simulink library "casper_library_scopes"  (Simulink 8.0)
settings: Solver=ode45  SolverMode=SingleTasking  StartTime=0.0  StopTime=10.0  RelTol=1e-3
libraries: xbsIndex_r4 x476, xps_library x33, casper_library_misc x13, casper_library_scopes x5, casper_library_flow_control x1, simulink x1
(part 2 of 5)

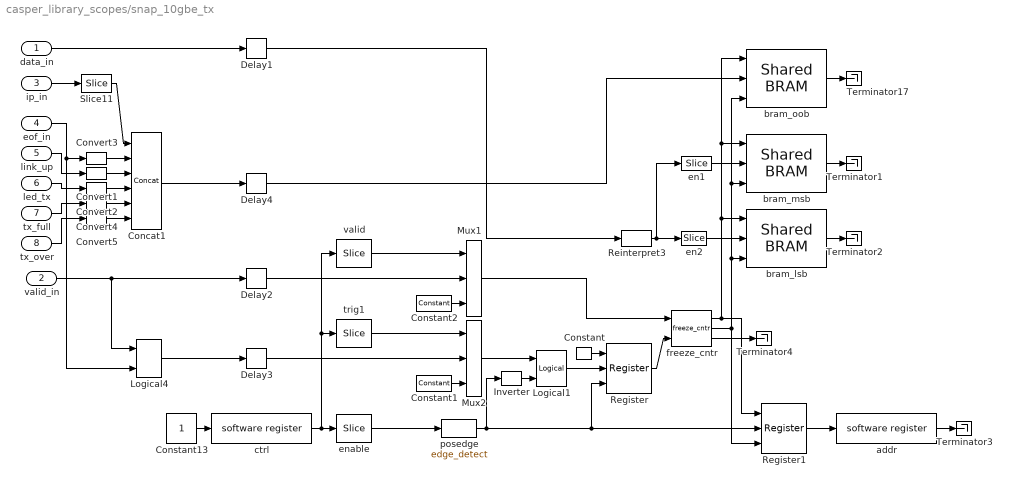
== system casper_library_scopes/snap_10gbe_tx ==
  data_in : Inport
  valid_in : Inport  Port=2
  ip_in : Inport  Port=3
  eof_in : Inport  Port=4
  link_up : Inport  Port=5
  led_tx : Inport  Port=6
  tx_full : Inport  Port=7
  tx_over : Inport  Port=8
  Concat1 : xbsIndex_r4/Concat  num_inputs=6  dbl_ovrd=off  block_type=concat
      settings: block_version=10.1.3
  Constant : xbsIndex_r4/Constant  const=1  gui_display_data_type=Fixed-point  arith_type=Boolean  n_bits=1  bin_pt=0  preci_type=Single  exp_width=8  frac_width=24  explicit_period=on  period=1  equ=P=C  opselect=C  inp2=PCIN>>17  opr=+  inp1=P  carry=CIN  dbl_ovrd=off  block_type=constant
  Constant1 : xbsIndex_r4/Constant  const=1  gui_display_data_type=Fixed-point  arith_type=Boolean  n_bits=1  bin_pt=0  preci_type=Single  exp_width=8  frac_width=24  explicit_period=on  period=1  equ=P=C  opselect=C  inp2=PCIN>>17  opr=+  inp1=P  carry=CIN  dbl_ovrd=off  block_type=constant
  Constant13 : Constant
  Constant2 : xbsIndex_r4/Constant  const=1  gui_display_data_type=Fixed-point  arith_type=Boolean  n_bits=1  bin_pt=0  preci_type=Single  exp_width=8  frac_width=24  explicit_period=on  period=1  equ=P=C  opselect=C  inp2=PCIN>>17  opr=+  inp1=P  carry=CIN  dbl_ovrd=off  block_type=constant
  Convert{1..5} (5 alike) : xbsIndex_r4/Convert  gui_display_data_type=Fixed-point  arith_type=Unsigned  n_bits=1  bin_pt=0  float_type=Single  exp_bits=8  fraction_bits=24  quantization=Truncate  overflow=Wrap  en=off  latency=0  dbl_ovrd=off  pipeline=off  block_type=convert
      settings: xl_area=[0, 0, 0, 0, 0, 0, 0]  block_version=10.1.3
  Delay{1..4} (4 alike) : xbsIndex_r4/Delay  rst=off  infoeditControl=Selection of Reset will increase slice count due to use of real FFs and instead of SRLs  en=off  latency=2  dbl_ovrd=off  reg_retiming=on  block_type=delay
      settings: xl_area=[0, 0, 0, 0, 0, 0, 0]
  Inverter : xbsIndex_r4/Inverter  en=off  latency=0  dbl_ovrd=off  block_type=inv
      settings: xl_area=[0, 0, 0, 0, 0, 0, 0]
  Logical1 : xbsIndex_r4/Logical  logical_function=AND  inputs=2  en=off  latency=0  precision=Full  arith_type=Unsigned  n_bits=8  bin_pt=2  align_bp=on  dbl_ovrd=off  block_type=logical
      settings: xl_area=[0, 0, 0, 0, 0, 0, 0]
  Logical4 : xbsIndex_r4/Logical  logical_function=AND  inputs=2  en=off  latency=0  precision=Full  arith_type=Unsigned  n_bits=8  bin_pt=2  align_bp=on  dbl_ovrd=off  block_type=logical
      settings: xl_area=[0, 0, 0, 0, 0, 0, 0]
  Mux1 : xbsIndex_r4/Mux  inputs=2  en=off  latency=0  precision=Full  arith_type="Signed  (2's comp)"  n_bits=8  bin_pt=2  quantization=Truncate  overflow=Wrap  dbl_ovrd=off  block_type=mux
      settings: xl_area=[0, 0, 0, 0, 0, 0, 0]
  Mux2 : xbsIndex_r4/Mux  inputs=2  en=off  latency=0  precision=Full  arith_type="Signed  (2's comp)"  n_bits=8  bin_pt=2  quantization=Truncate  overflow=Wrap  dbl_ovrd=off  block_type=mux
      settings: xl_area=[0, 0, 0, 0, 0, 0, 0]
  Register : xbsIndex_r4/Register  init=0  rst=on  en=on  dbl_ovrd=off  block_type=register
      settings: xl_area=[0, 0, 0, 0, 0, 0, 0]
  Register1 : xbsIndex_r4/Register  init=0  rst=on  en=on  dbl_ovrd=off  block_type=register
      settings: xl_area=[0, 0, 0, 0, 0, 0, 0]
  Reinterpret3 : xbsIndex_r4/Reinterpret  force_arith_type=on  arith_type=Unsigned  force_bin_pt=on  bin_pt=0  block_type=reinterpret
      settings: infoedit="Changes signal type without altering the binary representation.   You can changed the signal between signed and unsigned, and relocate the binary point.<P><P>Hardware notes: In hardware this block costs nothing.<P><P>Example:  Suppose the input is 6 bits wide, signed, with 2 fractional bits, and the output is forced to unsigned with 0 fractional bits.  Then an input of -2.0 (1110.00 in binary 2's complement) becomes an output of 56 (111000 in binary)."  block_version=10.1.3
  Slice11 : xbsIndex_r4/Slice  nbits=32-5  boolean_output=off  mode=Lower Bit Location + Width  bit1=0  base1=MSB of Input  bit0=0  base0=LSB of Input  dbl_ovrd=off  block_type=slice
      settings: infoedit="Extracts a given range of bits from each input sample and presents it at the output.  The output type is ordinarily unsigned with binary point at zero, but can be Boolean when the slice is one bit wide.<P><P>Hardware notes: In hardware this block costs nothing."  block_version=10.1.3
  Terminator{1..4,17} (5 alike) : Terminator
  addr : xps_library/software register  Tag=xps:sw_reg  numios=1  io_dir=To Processor  io_delay=0  sample_period=1  name1=reg  bitwidth1=32  arith_type1=Unsigned  bin_pt1=0
  bram_lsb : xps_library/Shared BRAM  Tag=xps:bram  arith_type=Unsigned  addr_width=nsamples  data_width=32  reg_prim_output=on  reg_core_output=on  optimization=Minimum_Area  data_bin_pt=0  init_vals=0  sample_rate=1
  bram_msb : xps_library/Shared BRAM  Tag=xps:bram  arith_type=Unsigned  addr_width=nsamples  data_width=32  reg_prim_output=on  reg_core_output=on  optimization=Minimum_Area  data_bin_pt=0  init_vals=0  sample_rate=1
  bram_oob : xps_library/Shared BRAM  Tag=xps:bram  arith_type=Unsigned  addr_width=nsamples  data_width=32  reg_prim_output=on  reg_core_output=on  optimization=Minimum_Area  data_bin_pt=0  init_vals=0  sample_rate=1
  ctrl : xps_library/software register  Tag=xps:sw_reg  numios=1  io_dir=From Processor  io_delay=0  sample_period=1  name1=reg  bitwidth1=32  arith_type1=Unsigned  bin_pt1=0
  en1 : xbsIndex_r4/Slice  nbits=32  boolean_output=off  mode=Lower Bit Location + Width  bit1=0  base1=LSB of Input  bit0=32  base0=LSB of Input  dbl_ovrd=off  block_type=slice
      settings: infoedit="Extracts a given range of bits from each input sample and presents it at the output.  The output type is ordinarily unsigned with binary point at zero, but can be Boolean when the slice is one bit wide.<P><P>Hardware notes: In hardware this block costs nothing."  block_version=10.1.3
  en2 : xbsIndex_r4/Slice  nbits=32  boolean_output=off  mode=Lower Bit Location + Width  bit1=0  base1=LSB of Input  bit0=0  base0=LSB of Input  dbl_ovrd=off  block_type=slice
      settings: infoedit="Extracts a given range of bits from each input sample and presents it at the output.  The output type is ordinarily unsigned with binary point at zero, but can be Boolean when the slice is one bit wide.<P><P>Hardware notes: In hardware this block costs nothing."  block_version=10.1.3
  enable : xbsIndex_r4/Slice  nbits=1  boolean_output=on  mode=Lower Bit Location + Width  bit1=0  base1=LSB of Input  bit0=0  base0=LSB of Input  dbl_ovrd=off  block_type=slice
      settings: infoedit="Extracts a given range of bits from each input sample and presents it at the output.  The output type is ordinarily unsigned with binary point at zero, but can be Boolean when the slice is one bit wide.<P><P>Hardware notes: In hardware this block costs nothing."  block_version=10.1.3
  freeze_cntr : casper_library_misc/freeze_cntr  CounterBits=nsamples
  posedge : casper_library_misc/edge_detect  edge=Rising  polarity=Active High  x_in=[0 0.08 0.08 0.16 0.16 0.24 0.24 0.32 0.32 0.4]  y_in="[-1 -1  1  1  1  1  1  1  1  1]"  x_out=[0.6 0.68 0.68 0.76 0.76 0.84 0.84 0.92 0.92 1]  y_out="[-1 -1  1  1 -1 -1 -1 -1 -1 -1]"
  trig1 : xbsIndex_r4/Slice  nbits=1  boolean_output=on  mode=Lower Bit Location + Width  bit1=0  base1=LSB of Input  bit0=1  base0=LSB of Input  dbl_ovrd=off  block_type=slice
      settings: infoedit="Extracts a given range of bits from each input sample and presents it at the output.  The output type is ordinarily unsigned with binary point at zero, but can be Boolean when the slice is one bit wide.<P><P>Hardware notes: In hardware this block costs nothing."  block_version=10.1.3
  valid : xbsIndex_r4/Slice  nbits=1  boolean_output=on  mode=Lower Bit Location + Width  bit1=0  base1=LSB of Input  bit0=2  base0=LSB of Input  dbl_ovrd=off  block_type=slice
      settings: infoedit="Extracts a given range of bits from each input sample and presents it at the output.  The output type is ordinarily unsigned with binary point at zero, but can be Boolean when the slice is one bit wide.<P><P>Hardware notes: In hardware this block costs nothing."  block_version=10.1.3
  wires:
  freeze_cntr/3 -> Terminator4/1
  addr/1 -> Terminator3/1
  bram_lsb/1 -> Terminator2/1
  bram_msb/1 -> Terminator1/1
  bram_oob/1 -> Terminator17/1
  Convert5/1 -> Concat1/6
  Convert4/1 -> Concat1/5
  Convert2/1 -> Concat1/4
  Convert1/1 -> Concat1/3
  Convert3/1 -> Concat1/2
  tx_over/1 -> Convert5/1
  tx_full/1 -> Convert4/1
  led_tx/1 -> Convert2/1
  link_up/1 -> Convert1/1
  eof_in/1 -> Logical4/2, Convert3/1
  Delay3/1 -> Mux2/2
  Delay2/1 -> Mux1/2
  valid_in/1 -> Logical4/1, Delay2/1
  Logical4/1 -> Delay3/1
  Delay4/1 -> bram_oob/2
  Delay1/1 -> Reinterpret3/1
  ip_in/1 -> Slice11/1
  data_in/1 -> Delay1/1
  Concat1/1 -> Delay4/1
  Slice11/1 -> Concat1/1
  freeze_cntr/1 -> bram_lsb/1, bram_msb/1, bram_oob/1, Register1/1
  Register/1 -> freeze_cntr/2
  Mux2/1 -> Logical1/1
  Inverter/1 -> Logical1/2
  Logical1/1 -> Register/2
  valid/1 -> Mux1/1
  trig1/1 -> Mux2/1
  Register1/1 -> addr/1
  Constant2/1 -> Mux1/3
  Mux1/1 -> freeze_cntr/1
  Constant1/1 -> Mux2/3
  Constant/1 -> Register/1
  posedge/1 -> Inverter/1, Register1/2, Register/3
  ctrl/1 -> trig1/1, valid/1, enable/1
  Constant13/1 -> ctrl/1
  freeze_cntr/2 -> bram_lsb/3, bram_msb/3, bram_oob/3, Register1/3
  enable/1 -> posedge/1
  Reinterpret3/1 -> en1/1, en2/1
  en1/1 -> bram_msb/2
  en2/1 -> bram_lsb/2

== system casper_library_scopes/snap_32n ==
  trig : Inport
  din : Inport  Port=2
  Constant : Constant  Value=0
  read_freeze : xps_library/software register  Tag=xps:sw_reg  numios=1  io_dir=From Processor  io_delay=0  sample_period=1  name1=reg  bitwidth1=32  arith_type1=Unsigned  bin_pt1=0
  sc0 : casper_library_scopes/sc  nsamples=11  offset=0
  sc1 : casper_library_scopes/sc  nsamples=11  offset=32
  sc2 : casper_library_scopes/sc  nsamples=11  offset=64
  sc3 : casper_library_scopes/sc  nsamples=11  offset=96
  wires:
  Constant/1 -> read_freeze/1
  trig/1 -> sc0/2, sc1/2, sc2/2, sc3/2
  din/1 -> sc0/1, sc1/1, sc2/1, sc3/1
  read_freeze/1 -> sc0/3, sc1/3, sc2/3, sc3/3

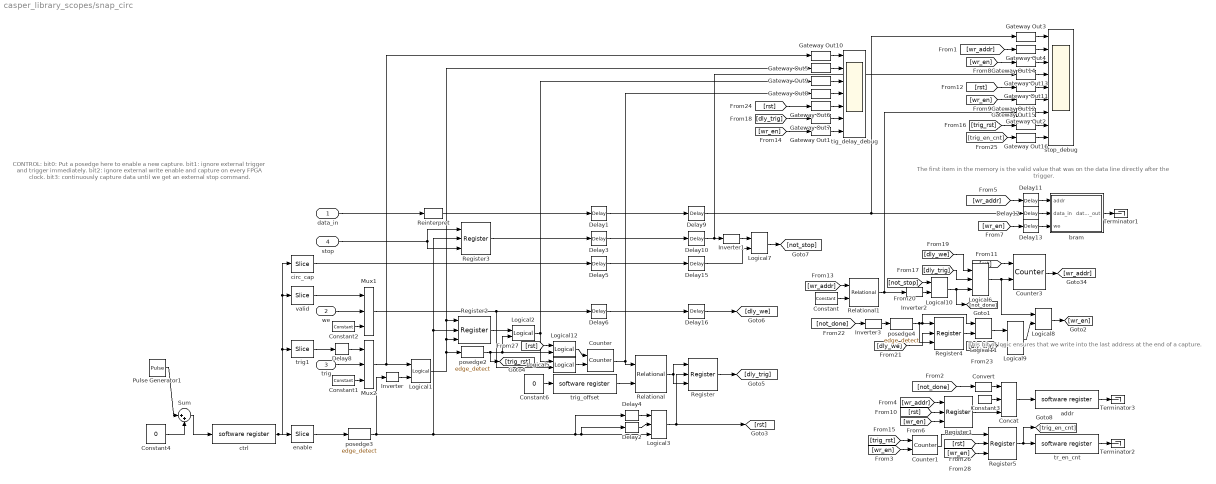
== system casper_library_scopes/snap_circ ==
  note: This bit of logic ensures that we
      | write into the last address
      | at the end of a capture.
  note: The first item in the memory
      | is the valid value that was on the
      | data line directly after the trigger.
  note: CONTROL:
      | bit0: Put a posedge here to enable a new capture.
      | bit1: ignore external trigger and trigger immediately.
      | bit2: ignore external write enable and capture on every FPGA clock.
      | bit3: continuously capture data until we get an external stop command.
  data_in : Inport
  we : Inport  Port=2
  trig : Inport  Port=3
  stop : Inport  Port=4
  Concat : xbsIndex_r4/Concat  num_inputs=3  dbl_ovrd=off  block_type=concat
      settings: block_version=10.1.3
  Constant : xbsIndex_r4/Constant  const=(2^nsamples)-1  gui_display_data_type=Fixed-point  arith_type=Unsigned  n_bits=nsamples  bin_pt=0  preci_type=Single  exp_width=8  frac_width=24  explicit_period=on  period=1  equ=P=C  opselect=C  inp2=PCIN>>17  opr=+  inp1=P  carry=CIN  dbl_ovrd=off  block_type=constant
  Constant1 : xbsIndex_r4/Constant  const=1  gui_display_data_type=Fixed-point  arith_type=Boolean  n_bits=1  bin_pt=0  preci_type=Single  exp_width=8  frac_width=24  explicit_period=on  period=1  equ=P=C  opselect=C  inp2=PCIN>>17  opr=+  inp1=P  carry=CIN  dbl_ovrd=off  block_type=constant
  Constant2 : xbsIndex_r4/Constant  const=1  gui_display_data_type=Fixed-point  arith_type=Boolean  n_bits=1  bin_pt=0  preci_type=Single  exp_width=8  frac_width=24  explicit_period=on  period=1  equ=P=C  opselect=C  inp2=PCIN>>17  opr=+  inp1=P  carry=CIN  dbl_ovrd=off  block_type=constant
  Constant3 : xbsIndex_r4/Constant  const=0  gui_display_data_type=Fixed-point  arith_type=Unsigned  n_bits=32-nsamples-1  bin_pt=0  preci_type=Single  exp_width=8  frac_width=24  explicit_period=on  period=1  equ=P=C  opselect=C  inp2=PCIN>>17  opr=+  inp1=P  carry=CIN  dbl_ovrd=off  block_type=constant
  Constant4 : Constant  Value=0
  Constant6 : Constant  Value=0
  Convert : xbsIndex_r4/Convert  gui_display_data_type=Fixed-point  arith_type=Unsigned  n_bits=1  bin_pt=0  float_type=Single  exp_bits=8  fraction_bits=24  quantization=Truncate  overflow=Wrap  en=off  latency=0  dbl_ovrd=off  pipeline=off  block_type=convert
      settings: block_version=10.1.3
  Counter : xbsIndex_r4/Counter  cnt_type=Free Running  cnt_to=Inf  operation=Up  start_count=0  cnt_by_val=1  arith_type=Unsigned  n_bits=32  bin_pt=0  load_pin=off  rst=on  en=on  explicit_period=on  period=1  dbl_ovrd=off  use_behavioral_HDL=off  implementation=Fabric  use_rpm=on  block_type=counter
      settings: xl_area=[0, 0, 0, 0, 0, 0, 0]
  Counter1 : xbsIndex_r4/Counter  cnt_type=Free Running  cnt_to=Inf  operation=Up  start_count=0  cnt_by_val=1  arith_type=Unsigned  n_bits=32  bin_pt=0  load_pin=off  rst=on  en=on  explicit_period=on  period=1  dbl_ovrd=off  use_behavioral_HDL=off  implementation=Fabric  use_rpm=on  block_type=counter
      settings: xl_area=[0, 0, 0, 0, 0, 0, 0]
  Counter3 : xbsIndex_r4/Counter  cnt_type=Free Running  cnt_to=1  operation=Up  start_count=0  cnt_by_val=1  arith_type=Unsigned  n_bits=nsamples  bin_pt=0  load_pin=off  rst=on  en=on  explicit_period=on  period=1  dbl_ovrd=off  use_behavioral_HDL=off  implementation=Fabric  use_rpm=on  block_type=counter
      settings: xl_area=[0, 0, 0, 0, 0, 0, 0]
  Delay{1,3..6,9..13,15..16} (12 alike) : xbsIndex_r4/Delay  rst=off  infoeditControl=Selection of Reset will increase slice count due to use of real FFs and instead of SRLs  en=off  latency=1  dbl_ovrd=off  reg_retiming=on  block_type=delay
      settings: xl_area=[0, 0, 0, 0, 0, 0, 0]
  Delay2 : xbsIndex_r4/Delay  rst=off  infoeditControl=Selection of Reset will increase slice count due to use of real FFs and instead of SRLs  en=off  latency=2  dbl_ovrd=off  reg_retiming=on  block_type=delay
      settings: xl_area=[0, 0, 0, 0, 0, 0, 0]
  Delay8 : xbsIndex_r4/Delay  rst=off  infoeditControl=Selection of Reset will increase slice count due to use of real FFs and instead of SRLs  en=off  latency=3  dbl_ovrd=off  reg_retiming=on  block_type=delay
      settings: xl_area=[0, 0, 0, 0, 0, 0, 0]
  Gateway Out{1..16} (16 alike) : xbsIndex_r4/Gateway Out  inherit_from_input=off  hdl_port=off  timing_constraint=None  locs_specified=off  LOCs={}  UseAsDAC=off  DACChannel='1'  block_type=gatewayout
      settings: infoedit="Gateway out block.  Converts Xilinx fixed point inputs into ouputs of type Simulink integer, double, or fixed point.<P><P>Hardware notes:  In hardware these blocks become top level output ports or are discarded, depending on how they are configured."  xl_area=[0, 0, 0, 0, 0, 0, 0]  block_version=10.1.3
  Inverter{,1..3} (4 alike) : xbsIndex_r4/Inverter  en=off  latency=0  dbl_ovrd=off  block_type=inv
      settings: xl_area=[0, 0, 0, 0, 0, 0, 0]
  Logical{1,5,7,9} (4 alike) : xbsIndex_r4/Logical  logical_function=AND  inputs=2  en=off  latency=0  precision=Full  arith_type=Unsigned  n_bits=8  bin_pt=2  align_bp=on  dbl_ovrd=off  block_type=logical
      settings: xl_area=[0, 0, 0, 0, 0, 0, 0]
  Logical{2,8,10..12} (5 alike) : xbsIndex_r4/Logical  logical_function=OR  inputs=2  en=off  latency=0  precision=Full  arith_type=Unsigned  n_bits=8  bin_pt=2  align_bp=on  dbl_ovrd=off  block_type=logical
      settings: xl_area=[0, 0, 0, 0, 0, 0, 0]
  Logical3 : xbsIndex_r4/Logical  logical_function=OR  inputs=3  en=off  latency=0  precision=Full  arith_type=Unsigned  n_bits=8  bin_pt=2  align_bp=on  dbl_ovrd=off  block_type=logical
      settings: xl_area=[0, 0, 0, 0, 0, 0, 0]
  Logical6 : xbsIndex_r4/Logical  logical_function=AND  inputs=3  en=off  latency=0  precision=Full  arith_type=Unsigned  n_bits=8  bin_pt=2  align_bp=on  dbl_ovrd=off  block_type=logical
      settings: xl_area=[0, 0, 0, 0, 0, 0, 0]
  Mux1 : xbsIndex_r4/Mux  inputs=2  en=off  latency=0  precision=Full  arith_type="Signed  (2's comp)"  n_bits=8  bin_pt=2  quantization=Truncate  overflow=Wrap  dbl_ovrd=off  block_type=mux
      settings: xl_area=[0, 0, 0, 0, 0, 0, 0]
  Mux2 : xbsIndex_r4/Mux  inputs=2  en=off  latency=0  precision=Full  arith_type="Signed  (2's comp)"  n_bits=8  bin_pt=2  quantization=Truncate  overflow=Wrap  dbl_ovrd=off  block_type=mux
      settings: xl_area=[0, 0, 0, 0, 0, 0, 0]
  Pulse Generator1 : DiscretePulseGenerator  Period=2^(nsamples+2)  PulseWidth=2
  Register{,1..5} (6 alike) : xbsIndex_r4/Register  init=0  rst=on  en=on  dbl_ovrd=off  block_type=register
      settings: xl_area=[0, 0, 0, 0, 0, 0, 0]
  Reinterpret : xbsIndex_r4/Reinterpret  force_arith_type=on  arith_type=Unsigned  force_bin_pt=on  bin_pt=0  block_type=reinterpret
      settings: infoedit="Changes signal type without altering the binary representation.   You can changed the signal between signed and unsigned, and relocate the binary point.<P><P>Hardware notes: In hardware this block costs nothing.<P><P>Example:  Suppose the input is 6 bits wide, signed, with 2 fractional bits, and the output is forced to unsigned with 0 fractional bits.  Then an input of -2.0 (1110.00 in binary 2's complement) becomes an output of 56 (111000 in binary)."  block_version=10.1.3
  Relational : xbsIndex_r4/Relational  mode=a>b  en=off  latency=0  dbl_ovrd=off  block_type=relational
      settings: xl_area=[0, 0, 0, 0, 0, 0, 0]  block_version=10.1.3
  Relational1 : xbsIndex_r4/Relational  mode=a>=b  en=off  latency=0  dbl_ovrd=off  block_type=relational
      settings: xl_area=[0, 0, 0, 0, 0, 0, 0]  block_version=10.1.3
  Sum : Sum  Inputs=|++
  Terminator1 : Terminator
  Terminator2 : Terminator
  Terminator3 : Terminator
  addr : xps_library/software register  Tag=xps:sw_reg  mode=one value  io_dir=To Processor  io_delay=0  sample_period=1  names=reg  bitwidths=32  arith_types=0  bin_pts=0  show_format=off
      settings: AttributesFormatString=1output
  bram : Subsystem  Tag=xps:bram  AncestorBlock=xps_library/Shared BRAM  mask{arith_type=Unsigned, addr_width=nsamples, data_width=32, reg_prim_output=on, reg_core_output=on, optimization=Minimum_Area, data_bin_pt=0, init_vals=0, sample_rate=1}
      mask prompts: arith_type "Output Data Type"; addr_width "Address width"; data_width "Data Width"; reg_prim_output "Register Primitive Output"; reg_core_output "Register Core Output"; data_bin_pt "Data Binary Point"; init_vals "Initial values (simulation only)"; sample_rate "Sample rate"
      mask init:
      | shared_bram_mask;
      mask TypeOptions arith_type: Unsigned | Signed  (2's comp)
      mask TypeOptions data_width: 8 | 16 | 32 | 64 | 128
      mask TypeOptions optimization: Minimum_Area | Low_Power
  circ_cap : xbsIndex_r4/Slice  nbits=1  boolean_output=on  mode=Lower Bit Location + Width  bit1=0  base1=LSB of Input  bit0=3  base0=LSB of Input  dbl_ovrd=off  block_type=slice
      settings: infoedit="Extracts a given range of bits from each input sample and presents it at the output.  The output type is ordinarily unsigned with binary point at zero, but can be Boolean when the slice is one bit wide.<P><P>Hardware notes: In hardware this block costs nothing."  block_version=10.1.3
  ctrl : xps_library/software register  Tag=xps:sw_reg  mode=one value  io_dir=From Processor  io_delay=0  sample_period=1  names=reg  bitwidths=32  arith_types=0  bin_pts=0  show_format=off
      settings: AttributesFormatString=1input
  enable : xbsIndex_r4/Slice  nbits=1  boolean_output=on  mode=Lower Bit Location + Width  bit1=0  base1=LSB of Input  bit0=0  base0=LSB of Input  dbl_ovrd=off  block_type=slice
      settings: infoedit="Extracts a given range of bits from each input sample and presents it at the output.  The output type is ordinarily unsigned with binary point at zero, but can be Boolean when the slice is one bit wide.<P><P>Hardware notes: In hardware this block costs nothing."  block_version=10.1.3
  posedge2 : casper_library_misc/edge_detect  edge=Rising  polarity=Active High  x_in=[0 0.08 0.08 0.16 0.16 0.24 0.24 0.32 0.32 0.4]  y_in="[-1 -1  1  1  1  1  1  1  1  1]"  x_out=[0.6 0.68 0.68 0.76 0.76 0.84 0.84 0.92 0.92 1]  y_out="[-1 -1  1  1 -1 -1 -1 -1 -1 -1]"
  posedge3 : casper_library_misc/edge_detect  edge=Rising  polarity=Active High  x_in=[0 0.08 0.08 0.16 0.16 0.24 0.24 0.32 0.32 0.4]  y_in="[-1 -1  1  1  1  1  1  1  1  1]"  x_out=[0.6 0.68 0.68 0.76 0.76 0.84 0.84 0.92 0.92 1]  y_out="[-1 -1  1  1 -1 -1 -1 -1 -1 -1]"
  posedge4 : casper_library_misc/edge_detect  edge=Rising  polarity=Active High  x_in=[0 0.08 0.08 0.16 0.16 0.24 0.24 0.32 0.32 0.4]  y_in="[-1 -1  1  1  1  1  1  1  1  1]"  x_out=[0.6 0.68 0.68 0.76 0.76 0.84 0.84 0.92 0.92 1]  y_out="[-1 -1  1  1 -1 -1 -1 -1 -1 -1]"
  stop_debug : Scope  NumInputPorts=9
      settings: YMin=2.72014e+008~0~0~-5~-5~-5~-5~-5~-5  YMax=3.00648e+008~110~1~5~5~5~5~5~5  SaveName=ScopeData12
  tig_delay_debug : Scope  NumInputPorts=7
      settings: YMin=2.72014e+008~0~0~-5~-5~-5~-5  YMax=3.00648e+008~110~1~5~5~5~5  SaveName=ScopeData16
  tr_en_cnt : xps_library/software register  Tag=xps:sw_reg  mode=one value  io_dir=To Processor  io_delay=0  sample_period=1  names=reg  bitwidths=32  arith_types=0  bin_pts=0  show_format=off
      settings: AttributesFormatString=1output
  trig1 : xbsIndex_r4/Slice  nbits=1  boolean_output=on  mode=Lower Bit Location + Width  bit1=0  base1=LSB of Input  bit0=1  base0=LSB of Input  dbl_ovrd=off  block_type=slice
      settings: infoedit="Extracts a given range of bits from each input sample and presents it at the output.  The output type is ordinarily unsigned with binary point at zero, but can be Boolean when the slice is one bit wide.<P><P>Hardware notes: In hardware this block costs nothing."  block_version=10.1.3
  trig_offset : xps_library/software register  Tag=xps:sw_reg  mode=one value  io_dir=From Processor  io_delay=0  sample_period=1  names=reg  bitwidths=32  arith_types=0  bin_pts=0  show_format=off
      settings: AttributesFormatString=1input
  valid : xbsIndex_r4/Slice  nbits=1  boolean_output=on  mode=Lower Bit Location + Width  bit1=0  base1=LSB of Input  bit0=2  base0=LSB of Input  dbl_ovrd=off  block_type=slice
      settings: infoedit="Extracts a given range of bits from each input sample and presents it at the output.  The output type is ordinarily unsigned with binary point at zero, but can be Boolean when the slice is one bit wide.<P><P>Hardware notes: In hardware this block costs nothing."  block_version=10.1.3
  wires:
  Delay6/1 -> Delay16/1
  Delay5/1 -> Delay15/1
  Delay3/1 -> Delay10/1
  Delay1/1 -> Delay9/1
  posedge2/1 -> [trig_rst], Logical12/2, Logical2/2
  [rst] -> Logical12/1
  Logical12/1 -> Counter/1
  Register5/1 -> [trig_en_cnt], tr_en_cnt/1
  [rst] -> Register5/2
  [wr_en] -> Register5/3
  Counter1/1 -> Register5/1
  Gateway Out16/1 -> stop_debug/9
  [trig_en_cnt] -> Gateway Out16/1
  Delay8/1 -> Mux2/1
  [rst] -> Gateway Out6/1
  Register4/1 -> Logical11/2
  Logical11/1 -> Logical9/1
  Logical9/1 -> Logical8/2
  [dly_we] -> Logical9/2
  [dly_we] -> Register4/2
  posedge4/1 -> Logical11/1, Register4/1, Register4/3
  Inverter3/1 -> posedge4/1
  [not_done] -> Inverter3/1
  Logical8/1 -> [wr_en]
  [not_stop] -> Logical10/1
  Logical7/1 -> [not_stop]
  [dly_trig] -> Logical6/2
  [dly_we] -> Logical6/1
  Delay16/1 -> [dly_we]
  [dly_trig] -> Gateway Out7/1
  Register/1 -> [dly_trig]
  [trig_rst] -> Gateway Out15/1
  Gateway Out15/1 -> stop_debug/8
  [trig_rst] -> Counter1/1
  [wr_en] -> Gateway Out1/1
  [wr_addr] -> Relational1/1
  Relational1/1 -> Inverter2/1, Gateway Out2/1
  [rst] -> Gateway Out11/1
  [rst] -> Counter3/1
  [rst] -> Register1/2
  [wr_en] -> Gateway Out12/1
  [wr_en] -> Gateway Out14/1
  [wr_en] -> Delay13/1
  [wr_en] -> Register1/3
  [wr_addr] -> Register1/1
  [wr_en] -> Counter1/2
  [not_done] -> Convert/1
  [wr_addr] -> Gateway Out4/1
  [wr_addr] -> Delay11/1
  Register1/1 -> Concat/3
  Logical5/1 -> Counter/2
  Delay15/1 -> Logical7/2
  Delay10/1 -> Gateway Out13/1, Inverter1/1
  Delay9/1 -> Gateway Out3/1, Delay12/1
  bram/1(data_out) -> Terminator1/1
  addr/1 -> Terminator3/1
  tr_en_cnt/1 -> Terminator2/1
  Constant3/1 -> Concat/2
  Convert/1 -> Concat/1
  circ_cap/1 -> Delay5/1
  stop/1 -> Register3/3, Register3/1
  Concat/1 -> addr/1
  Delay13/1 -> bram/3(we)
  Delay12/1 -> bram/2(data_in)
  Delay11/1 -> bram/1(addr)
  Inverter2/1 -> Logical10/2
  Logical10/1 -> [not_done], Logical6/3
  Logical3/1 -> [rst], Register/2
  Gateway Out2/1 -> stop_debug/7
  Gateway Out12/1 -> stop_debug/6
  Gateway Out3/1 -> stop_debug/1
  Gateway Out11/1 -> stop_debug/5
  Gateway Out13/1 -> stop_debug/4
  Gateway Out4/1 -> stop_debug/2
  Gateway Out14/1 -> stop_debug/3
  Inverter1/1 -> Logical7/1
  Register3/1 -> Delay3/1
  Constant/1 -> Relational1/2
  Counter3/1 -> [wr_addr]
  Logical6/1 -> Logical8/1, Counter3/2
  Reinterpret/1 -> Delay1/1
  Gateway Out1/1 -> tig_delay_debug/7
  Gateway Out7/1 -> tig_delay_debug/6
  Gateway Out10/1 -> tig_delay_debug/1
  Gateway Out6/1 -> tig_delay_debug/5
  Gateway Out8/1 -> tig_delay_debug/4
  Gateway Out5/1 -> tig_delay_debug/2
  Gateway Out9/1 -> tig_delay_debug/3
  Delay2/1 -> Logical3/2
  Counter/1 -> Relational/1, Gateway Out8/1
  Logical2/1 -> Gateway Out9/1, Logical5/1
  Relational/1 -> Register/1, Register/3
  trig_offset/1 -> Relational/2
  Constant6/1 -> trig_offset/1
  Delay4/1 -> Logical3/1
  Register2/1 -> Logical2/1
  Logical1/1 -> posedge2/1, Register2/3, Gateway Out5/1, Register2/1
  posedge3/1 -> Register3/2, Register2/2, Logical3/3, Delay2/1, Delay4/1, Inverter/1
  Mux1/1 -> Delay6/1, Logical5/2
  Inverter/1 -> Logical1/2
  Mux2/1 -> Gateway Out10/1, Logical1/1
  Pulse Generator1/1 -> Sum/1
  Sum/1 -> ctrl/1
  Constant4/1 -> Sum/2
  trig/1 -> Mux2/2
  enable/1 -> posedge3/1
  ctrl/1 -> enable/1, circ_cap/1, valid/1, trig1/1
  Constant1/1 -> Mux2/3
  we/1 -> Mux1/2
  Constant2/1 -> Mux1/3
  trig1/1 -> Delay8/1
  valid/1 -> Mux1/1
  data_in/1 -> Reinterpret/1

== system casper_library_scopes/snapshot ==
  note: Value on vin
      | aligned with
      | first sample on
      | din captured
  note: Number of valid
      | data samples to
      | skip after trigger
      | before starting
      | capture
  note: Number of
      | bytes in
      | buffer and
      | done bit
  note: Offset in vector
      | from first element
      | captured, used
      | during circular capture
  note: ctrl:
      | bit0: Put a posedge here
      |         to enable a new capture.
      | bit1: ignore external trigger
      |         and trigger immediately.
      | bit2: ignore external write
      |         enable and capture on
      |         every FPGA clock.
      | bit3: continuously capture
      |         data until we get an
      |         external stop command.
  note: Delay start
      | of capture
  note: Generate stop
      | when in circular
      | capture mode
  din : Inport
  we : Inport  Port=2
  trig : Inport  Port=3
  stop : Inport  Port=4
  vin : Inport  Port=5
  add_del : xbsIndex_r4/Delay  rst=off  infoeditControl=Selection of Reset will increase slice count due to use of real FFs and instead of SRLs  en=off  latency=1  dbl_ovrd=off  reg_retiming=on  block_type=delay
      settings: block_version=11.4
  add_gen : Subsystem  mask{counter_size=32, increment=4, nsamples=10, burst_size=0, use_dsp48=on}
      mask prompts: counter_size "Address counter size (2^?)"; increment "Address counter increment"; nsamples "Number of samples (2^?)"; burst_size "Burst size (2^?)"; use_dsp48 "dsp48 counter/s"
      mask init:
      | set_param(gcb,'LinkStatus','inactive');
      | if strcmp(use_dsp48,'on'),
      |     set_param([gcb,'/add_gen'],'implementation','DSP48');
      | else
      |     set_param([gcb,'/add_gen'],'implementation','Fabric');
      | end
  basic_ctrl : Subsystem  mask{dram=off, data_width=32}
      mask prompts: data_width "data width"
      mask init:
      | set_param(gcb,'LinkStatus','inactive');
      | set_param([gcb,'/dram_munge'], 'dram', dram);
  bram : Subsystem  Tag=xps:bram  AncestorBlock=xps_library/Shared BRAM  mask{arith_type=Unsigned, addr_width=10, data_width=32, reg_prim_output=on, reg_core_output=on, optimization=Minimum_Area, data_bin_pt=0, init_vals=[0:2^10-1], sample_rate=1}
      mask prompts: arith_type "Output Data Type"; addr_width "Address width"; data_width "Data Width"; reg_prim_output "Register Primitive Output"; reg_core_output "Register Core Output"; data_bin_pt "Data Binary Point"; init_vals "Initial values (simulation only)"; sample_rate "Sample rate"
      mask init:
      | shared_bram_mask;
      mask TypeOptions arith_type: Unsigned | Signed  (2's comp)
      mask TypeOptions data_width: 8 | 16 | 32 | 64 | 128
      mask TypeOptions optimization: Minimum_Area | Low_Power
  cast : xbsIndex_r4/Convert  gui_display_data_type=Fixed-point  arith_type=Unsigned  n_bits=32  bin_pt=0  float_type=Single  exp_bits=8  fraction_bits=24  quantization=Truncate  overflow=Wrap  en=off  latency=0  dbl_ovrd=off  pipeline=off  block_type=convert
      settings: block_version=11.4
  const0 : Constant  Value=0
  const1 : Constant  Value=10
  ctrl : xps_library/software register  Tag=xps:sw_reg  io_dir=From Processor  io_delay=0  sample_period=1  names=reg  bitwidths=32  bin_pts=0  arith_types=0  sim_port=on  show_format=on
      settings: AttributesFormatString=1input:uf32.0
  dat_del : xbsIndex_r4/Delay  rst=off  infoeditControl=Selection of Reset will increase slice count due to use of real FFs and instead of SRLs  en=off  latency=1  dbl_ovrd=off  reg_retiming=on  block_type=delay
      settings: block_version=11.4
  delay : Subsystem  mask{use_dsp48=on, word_size=4}
      mask prompts: use_dsp48 "dsp48 counter/s"; word_size "word byte size?"
      mask init:
      | set_param(gcb,'LinkStatus','inactive');
      | if strcmp(use_dsp48,'on'),
      |     set_param([gcb,'/counter'],'implementation','DSP48');
      | else
      |     set_param([gcb,'/counter'],'implementation','Fabric');
      | end
  g_tr_en_cnt : Terminator
  gbram : Terminator
  gstatus : Terminator
  gval : Terminator
  ri : xbsIndex_r4/Reinterpret  force_arith_type=on  arith_type=Unsigned  force_bin_pt=on  bin_pt=0  block_type=reinterpret
      settings: infoedit="Changes signal type without altering the binary representation.   You can changed the signal between signed and unsigned, and relocate the binary point.<br><br>Hardware notes: In hardware this block costs nothing.<br><br>Example:  Suppose the input is 6 bits wide, signed, with 2 fractional bits, and the output is forced to unsigned with 0 fractional bits.  Then an input of -2.0 (1110.00 in binary 2's complement) becomes an output of 56 (111000 in binary)."
  status : xps_library/software register  Tag=xps:sw_reg  io_dir=To Processor  io_delay=0  sample_period=1  names=reg  bitwidths=32  bin_pts=0  arith_types=0  sim_port=on  show_format=on
      settings: AttributesFormatString=1output:uf32.0
  stop_gen : Subsystem
  tr_en_cnt : xps_library/software register  Tag=xps:sw_reg  io_dir=To Processor  io_delay=0  sample_period=1  names=reg  bitwidths=32  bin_pts=0  arith_types=0  sim_port=on  show_format=on
      settings: AttributesFormatString=1output:uf32.0
  trig_offset : xps_library/software register  Tag=xps:sw_reg  io_dir=From Processor  io_delay=0  sample_period=1  names=reg  bitwidths=32  bin_pts=0  arith_types=0  sim_port=on  show_format=on
      settings: AttributesFormatString=1input:uf32.0
  val : xps_library/software register  Tag=xps:sw_reg  io_dir=To Processor  io_delay=0  sample_period=1  names=reg  bitwidths=32  bin_pts=0  arith_types=0  sim_port=on  show_format=on
      settings: AttributesFormatString=1output:uf32.0
  we_del : xbsIndex_r4/Delay  rst=off  infoeditControl=Selection of Reset will increase slice count due to use of real FFs and instead of SRLs  en=off  latency=1  dbl_ovrd=off  reg_retiming=on  block_type=delay
      settings: block_version=11.4
  wires:
  bram/1(data_out) -> gbram/1
  we_del/1 -> bram/3(we)
  dat_del/1 -> bram/2(data_in)
  add_del/1 -> bram/1(addr)
  add_gen/4(we_o) -> we_del/1
  add_gen/3(dout) -> dat_del/1
  add_gen/2(add) -> add_del/1
  add_gen/6(en_cnt) -> tr_en_cnt/1
  val/1 -> gval/1
  add_gen/1(vout) -> val/1
  vin/1 -> basic_ctrl/1(vin)
  status/1 -> gstatus/1
  add_gen/5(status) -> status/1
  stop_gen/6(inito) -> add_gen/6(init)
  stop_gen/5(cont) -> add_gen/5(cont)
  stop_gen/4(go) -> add_gen/4(go)
  stop_gen/3(weo) -> add_gen/3(we)
  stop_gen/2(dout) -> add_gen/2(din)
  stop_gen/1(vout) -> add_gen/1(vin)
  tr_en_cnt/1 -> g_tr_en_cnt/1
  delay/6(del_init) -> stop_gen/6(init)
  delay/5(stop) -> stop_gen/5(stop)
  delay/4(del_go) -> stop_gen/4(goi)
  delay/3(we_o) -> stop_gen/3(wei)
  delay/2(dout) -> stop_gen/2(din)
  delay/1(vout) -> stop_gen/1(vin)
  trig_offset/1 -> delay/7(delay)
  basic_ctrl/6(init) -> delay/6(init)
  basic_ctrl/5(stop) -> delay/5(stopi)
  basic_ctrl/4(go) -> delay/4(go)
  basic_ctrl/3(we_o) -> delay/3(we)
  basic_ctrl/2(dout) -> delay/2(din)
  basic_ctrl/1(vout) -> delay/1(vin)
  const1/1 -> trig_offset/1
  ctrl/1 -> stop_gen/7(ctrl), basic_ctrl/5(ctrl)
  const0/1 -> ctrl/1
  stop/1 -> basic_ctrl/6(stopi)
  trig/1 -> basic_ctrl/4(trig)
  we/1 -> basic_ctrl/3(we)
  cast/1 -> basic_ctrl/2(din)
  ri/1 -> cast/1
  din/1 -> ri/1

== system casper_library_scopes/bitfield snapshot/buscreate ==
  in1 : Inport
  in2 : Inport  Port=2
  concatenate : xbsIndex_r4/Concat  num_inputs=2  dbl_ovrd=off  block_type=concat
  reinterpret1 : xbsIndex_r4/Reinterpret  force_arith_type=on  arith_type=Unsigned  force_bin_pt=on  bin_pt=0  block_type=reinterpret
  reinterpret2 : xbsIndex_r4/Reinterpret  force_arith_type=on  arith_type=Unsigned  force_bin_pt=on  bin_pt=0  block_type=reinterpret
  bus_out : Outport
  wires:
  reinterpret2/1 -> concatenate/2
  in2/1 -> reinterpret2/1
  reinterpret1/1 -> concatenate/1
  in1/1 -> reinterpret1/1
  concatenate/1 -> bus_out/1

== system casper_library_scopes/bitfield snapshot/extracreate ==
  in1 : Inport
  in2 : Inport  Port=2
  concatenate : xbsIndex_r4/Concat  num_inputs=2  dbl_ovrd=off  block_type=concat
  reinterpret1 : xbsIndex_r4/Reinterpret  force_arith_type=on  arith_type=Unsigned  force_bin_pt=on  bin_pt=0  block_type=reinterpret
      settings: infoedit="Changes signal type without altering the binary representation.   You can changed the signal between signed and unsigned, and relocate the binary point.<br><br>Hardware notes: In hardware this block costs nothing.<br><br>Example:  Suppose the input is 6 bits wide, signed, with 2 fractional bits, and the output is forced to unsigned with 0 fractional bits.  Then an input of -2.0 (1110.00 in binary 2's complement) becomes an output of 56 (111000 in binary)."
  reinterpret2 : xbsIndex_r4/Reinterpret  force_arith_type=on  arith_type=Unsigned  force_bin_pt=on  bin_pt=0  block_type=reinterpret
      settings: infoedit="Changes signal type without altering the binary representation.   You can changed the signal between signed and unsigned, and relocate the binary point.<br><br>Hardware notes: In hardware this block costs nothing.<br><br>Example:  Suppose the input is 6 bits wide, signed, with 2 fractional bits, and the output is forced to unsigned with 0 fractional bits.  Then an input of -2.0 (1110.00 in binary 2's complement) becomes an output of 56 (111000 in binary)."
  bus_out : Outport
  wires:
  reinterpret2/1 -> concatenate/2
  in2/1 -> reinterpret2/1
  reinterpret1/1 -> concatenate/1
  in1/1 -> reinterpret1/1
  concatenate/1 -> bus_out/1

== system casper_library_scopes/bitfield snapshot/ss ==
  note: Value on vin
      | aligned with
      | first sample on
      | din captured
  note: Number of valid
      | data samples to
      | skip after trigger
      | before starting
      | capture
  note: Number of
      | bytes in
      | buffer and
      | done bit
  note: Offset in vector
      | from first element
      | captured, used
      | during circular capture
  note: ctrl:
      | bit0: Put a posedge here
      |         to enable a new capture.
      | bit1: ignore external trigger
      |         and trigger immediately.
      | bit2: ignore external write
      |         enable and capture on
      |         every FPGA clock.
      | bit3: continuously capture
      |         data until we get an
      |         external stop command.
  note: Delay start
      | of capture
  note: Generate stop
      | when in circular
      | capture mode
  din : Inport
  we : Inport  Port=2
  trig : Inport  Port=3
  stop : Inport  Port=4
  vin : Inport  Port=5
  add_del : xbsIndex_r4/Delay  rst=off  infoeditControl=Selection of Reset will increase slice count due to use of real FFs and instead of SRLs  en=off  latency=1  dbl_ovrd=off  reg_retiming=on  block_type=delay
      settings: block_version=11.4
  add_gen : Subsystem  AncestorBlock=casper_library_scopes/snapshot/add_gen  mask{counter_size=32, increment=4, nsamples=10, burst_size=0, use_dsp48=on}
      mask prompts: counter_size "Address counter size (2^?)"; increment "Address counter increment"; nsamples "Number of samples (2^?)"; burst_size "Burst size (2^?)"; use_dsp48 "dsp48 counter/s"
      mask init:
      | set_param(gcb,'LinkStatus','inactive');
      | if strcmp(use_dsp48,'on'),
      |     set_param([gcb,'/add_gen'],'implementation','DSP48');
      | else
      |     set_param([gcb,'/add_gen'],'implementation','Fabric');
      | end
  basic_ctrl : Subsystem  AncestorBlock=casper_library_scopes/snapshot/basic_ctrl  mask{dram=off, data_width=32}
      mask prompts: data_width "data width"
      mask init:
      | set_param(gcb,'LinkStatus','inactive');
      | set_param([gcb,'/dram_munge'], 'dram', dram);
  bram : Subsystem  Tag=xps:bram  AncestorBlock=xps_library/Shared BRAM  mask{arith_type=Unsigned, addr_width=10, data_width=32, reg_prim_output=on, reg_core_output=on, optimization=Minimum_Area, data_bin_pt=0, init_vals=[0:2^10-1], sample_rate=1}
      mask prompts: arith_type "Output Data Type"; addr_width "Address width"; data_width "Data Width"; reg_prim_output "Register Primitive Output"; reg_core_output "Register Core Output"; data_bin_pt "Data Binary Point"; init_vals "Initial values (simulation only)"; sample_rate "Sample rate"
      mask init:
      | shared_bram_mask;
      mask TypeOptions arith_type: Unsigned | Signed  (2's comp)
      mask TypeOptions data_width: 8 | 16 | 32 | 64 | 128
      mask TypeOptions optimization: Minimum_Area | Low_Power
  cast : xbsIndex_r4/Convert  gui_display_data_type=Fixed-point  arith_type=Unsigned  n_bits=32  bin_pt=0  float_type=Single  exp_bits=8  fraction_bits=24  quantization=Truncate  overflow=Wrap  en=off  latency=0  dbl_ovrd=off  pipeline=off  block_type=convert
      settings: block_version=11.4
  const0 : Constant  Value=0
  const1 : Constant  Value=10
  ctrl : xps_library/software register  Tag=xps:sw_reg  io_dir=From Processor  io_delay=0  sample_period=1  names=reg  bitwidths=32  bin_pts=0  arith_types=0  sim_port=on  show_format=on
      settings: AttributesFormatString=1input:uf32.0
  dat_del : xbsIndex_r4/Delay  rst=off  infoeditControl=Selection of Reset will increase slice count due to use of real FFs and instead of SRLs  en=off  latency=1  dbl_ovrd=off  reg_retiming=on  block_type=delay
      settings: block_version=11.4
  delay : Subsystem  AncestorBlock=casper_library_scopes/snapshot/delay  mask{use_dsp48=on, word_size=4}
      mask prompts: use_dsp48 "dsp48 counter/s"; word_size "word byte size?"
      mask init:
      | set_param(gcb,'LinkStatus','inactive');
      | if strcmp(use_dsp48,'on'),
      |     set_param([gcb,'/counter'],'implementation','DSP48');
      | else
      |     set_param([gcb,'/counter'],'implementation','Fabric');
      | end
  g_tr_en_cnt : Terminator
  gbram : Terminator
  gstatus : Terminator
  gval : Terminator
  ri : xbsIndex_r4/Reinterpret  force_arith_type=on  arith_type=Unsigned  force_bin_pt=on  bin_pt=0  block_type=reinterpret
      settings: infoedit="Changes signal type without altering the binary representation.   You can changed the signal between signed and unsigned, and relocate the binary point.<br><br>Hardware notes: In hardware this block costs nothing.<br><br>Example:  Suppose the input is 6 bits wide, signed, with 2 fractional bits, and the output is forced to unsigned with 0 fractional bits.  Then an input of -2.0 (1110.00 in binary 2's complement) becomes an output of 56 (111000 in binary)."
  status : xps_library/software register  Tag=xps:sw_reg  io_dir=To Processor  io_delay=0  sample_period=1  names=reg  bitwidths=32  bin_pts=0  arith_types=0  sim_port=on  show_format=on
      settings: AttributesFormatString=1output:uf32.0
  stop_gen : casper_library_scopes/snapshot/stop_gen
  tr_en_cnt : xps_library/software register  Tag=xps:sw_reg  io_dir=To Processor  io_delay=0  sample_period=1  names=reg  bitwidths=32  bin_pts=0  arith_types=0  sim_port=on  show_format=on
      settings: AttributesFormatString=1output:uf32.0
  trig_offset : xps_library/software register  Tag=xps:sw_reg  io_dir=From Processor  io_delay=0  sample_period=1  names=reg  bitwidths=32  bin_pts=0  arith_types=0  sim_port=on  show_format=on
      settings: AttributesFormatString=1input:uf32.0
  val : xps_library/software register  Tag=xps:sw_reg  io_dir=To Processor  io_delay=0  sample_period=1  names=reg  bitwidths=32  bin_pts=0  arith_types=0  sim_port=on  show_format=on
      settings: AttributesFormatString=1output:uf32.0
  we_del : xbsIndex_r4/Delay  rst=off  infoeditControl=Selection of Reset will increase slice count due to use of real FFs and instead of SRLs  en=off  latency=1  dbl_ovrd=off  reg_retiming=on  block_type=delay
      settings: block_version=11.4
  wires:
  din/1 -> ri/1
  ri/1 -> cast/1
  cast/1 -> basic_ctrl/2(din)
  we/1 -> basic_ctrl/3(we)
  trig/1 -> basic_ctrl/4(trig)
  stop/1 -> basic_ctrl/6(stopi)
  const0/1 -> ctrl/1
  ctrl/1 -> basic_ctrl/5(ctrl), stop_gen/7
  const1/1 -> trig_offset/1
  basic_ctrl/1(vout) -> delay/1(vin)
  basic_ctrl/2(dout) -> delay/2(din)
  basic_ctrl/3(we_o) -> delay/3(we)
  basic_ctrl/4(go) -> delay/4(go)
  basic_ctrl/5(stop) -> delay/5(stopi)
  basic_ctrl/6(init) -> delay/6(init)
  trig_offset/1 -> delay/7(delay)
  delay/1(vout) -> stop_gen/1
  delay/2(dout) -> stop_gen/2
  delay/3(we_o) -> stop_gen/3
  delay/4(del_go) -> stop_gen/4
  delay/5(stop) -> stop_gen/5
  delay/6(del_init) -> stop_gen/6
  tr_en_cnt/1 -> g_tr_en_cnt/1
  stop_gen/1 -> add_gen/1(vin)
  stop_gen/2 -> add_gen/2(din)
  stop_gen/3 -> add_gen/3(we)
  stop_gen/4 -> add_gen/4(go)
  stop_gen/5 -> add_gen/5(cont)
  stop_gen/6 -> add_gen/6(init)
  add_gen/5(status) -> status/1
  status/1 -> gstatus/1
  vin/1 -> basic_ctrl/1(vin)
  add_gen/1(vout) -> val/1
  val/1 -> gval/1
  add_gen/6(en_cnt) -> tr_en_cnt/1
  add_gen/2(add) -> add_del/1
  add_gen/3(dout) -> dat_del/1
  add_gen/4(we_o) -> we_del/1
  add_del/1 -> bram/1(addr)
  dat_del/1 -> bram/2(data_in)
  we_del/1 -> bram/3(we)
  bram/1(data_out) -> gbram/1

== system casper_library_scopes/snap_circ/bram ==
  addr : Inport
  data_in : Inport  Port=2
  we : Inport  Port=3
  calc_add : Subsystem  mask{data_width=32, addr_width=10, sample_rate=sample_rate}
      mask prompts: data_width "data width"; addr_width "address width"; sample_rate "sample rate"
  casper_library_scopes_snap_circ_bram_addr : xbsIndex_r4/Gateway Out  inherit_from_input=off  hdl_port=on  timing_constraint=None  locs_specified=off  LOCs={'A5','B9','A9','C1','A3','G6','E9','A6','A7','A8','B8','B1','B3','D9','B5','B4','B6','C2'}  UseAsDAC=off  DACChannel='1'  block_type=gatewayout
      settings: infoedit="Gateway out block.  Converts Xilinx fixed point inputs into ouputs of type Simulink integer, double, or fixed point.<P><P>Hardware notes:  In hardware these blocks become top level output ports or are discarded, depending on how they are configured."  xl_area=[0, 0, 0, 0, 0, 0, 0]  sginterface={'Nallatech'=>{'xdspkit'=>{'non_memory_mapped_port'=>'uprev_Shared_BRAM_addr'}},'Xilinx'=>{'jtaghwcosim'=>{'non_memory_mapped_port'=>'uprev_Shared_BRAM_addr'},'xdspkit'=>{'non_memory_mapped_port'=>'uprev_Shared_BRAM_addr'}}}
  casper_library_scopes_snap_circ_bram_data_in : xbsIndex_r4/Gateway Out  inherit_from_input=off  hdl_port=on  timing_constraint=None  locs_specified=off  LOCs={'B21','B22','A22','B23','B19','C19','A20','A21','A23','B24','A24','A25','E18','D18','C18','B18'}  UseAsDAC=off  DACChannel='1'  block_type=gatewayout
      settings: infoedit="Gateway out block.  Converts Xilinx fixed point inputs into ouputs of type Simulink integer, double, or fixed point.<P><P>Hardware notes:  In hardware these blocks become top level output ports or are discarded, depending on how they are configured."  xl_area=[0, 0, 0, 0, 0, 0, 0]  sginterface={'Nallatech'=>{'xdspkit'=>{'non_memory_mapped_port'=>'uprev_Shared_BRAM_data_in'}},'Xilinx'=>{'jtaghwcosim'=>{'non_memory_mapped_port'=>'uprev_Shared_BRAM_data_in'},'xdspkit'=>{'non_memory_mapped_port'=>'uprev_Shared_BRAM_data_in'}}}
  casper_library_scopes_snap_circ_bram_data_out : xbsIndex_r4/Gateway In  gui_display_data_type=Fixed-point  arith_type=Unsigned  n_bits=32  bin_pt=0  preci_type=Single  exp_width=8  frac_width=24  quantization=Truncate  overflow=Wrap  period=sample_rate  dbl_ovrd=off  timing_constraint=None  locs_specified=off  LOCs={}  UseAsADC=off  ADCChannel='1'  inherit_from_input=off  hdl_port=on  block_type=gatewayin
      settings: xl_area=[0, 0, 0, 0, 0, 0, 0]
  casper_library_scopes_snap_circ_bram_we : xbsIndex_r4/Gateway Out  inherit_from_input=off  hdl_port=on  timing_constraint=None  locs_specified=off  LOCs={'A14'}  UseAsDAC=off  DACChannel='1'  block_type=gatewayout
      settings: infoedit="Gateway out block.  Converts Xilinx fixed point inputs into ouputs of type Simulink integer, double, or fixed point.<P><P>Hardware notes:  In hardware these blocks become top level output ports or are discarded, depending on how they are configured."  xl_area=[0, 0, 0, 0, 0, 0, 0]
  convert_addr : xbsIndex_r4/Convert  gui_display_data_type=Fixed-point  arith_type=Unsigned  n_bits=addr_width  bin_pt=0  float_type=Single  exp_bits=8  fraction_bits=24  quantization=Truncate  overflow=Wrap  en=off  latency=0  dbl_ovrd=off  pipeline=off  block_type=convert
      settings: xl_area=[0, 0, 0, 0, 0, 0, 0]
  convert_din1 : xbsIndex_r4/Convert  gui_display_data_type=Fixed-point  arith_type=Unsigned  n_bits=32  bin_pt=0  float_type=Single  exp_bits=8  fraction_bits=24  quantization=Truncate  overflow=Wrap  en=off  latency=0  dbl_ovrd=off  pipeline=off  block_type=convert
      settings: xl_area=[0, 0, 0, 0, 0, 0, 0]
  convert_we : xbsIndex_r4/Convert  gui_display_data_type=Fixed-point  arith_type=Unsigned  n_bits=1  bin_pt=0  float_type=Single  exp_bits=8  fraction_bits=24  quantization=Truncate  overflow=Wrap  en=off  latency=0  dbl_ovrd=off  pipeline=off  block_type=convert
      settings: xl_area=[0, 0, 0, 0, 0, 0, 0]
  mem : Subsystem
  munge_in : Subsystem  AncestorBlock=casper_library_flow_control/munge  mask(munge){divisions=1, div_size=32, order=[0], arith_type_out=Unsigned, bin_pt_out=0}
      mask prompts: divisions "Number of divisions"; div_size "Division size (bits)"; order "Division packing order"; arith_type_out "Output arithmetic type"; bin_pt_out "Output binary point"
      mask help: Splits an input bus into the specified number of divisions and then recombines them in the order specified (most significant division = 0,least = number divisions-1)
      mask init:
      | munge_init(gcb, ...
      |     'divisions', divisions, ...
      |     'div_size', div_size, ...
      |     'order', order, ...
      |     'arith_type_out', arith_type_out, ...
      |     'bin_pt_out', bin_pt_out);
      settings: AttributesFormatString=|
      | split:32
      | join:0
      | Unsigned [32,0]
      mask TypeOptions arith_type_out: Unsigned | Signed  (2's comp) | Floating-point
  munge_out : Subsystem  AncestorBlock=casper_library_flow_control/munge  mask(munge){divisions=1, div_size=32, order=[0], arith_type_out=Unsigned, bin_pt_out=0}
      mask prompts: divisions "Number of divisions"; div_size "Division size (bits)"; order "Division packing order"; arith_type_out "Output arithmetic type"; bin_pt_out "Output binary point"
      mask help: Splits an input bus into the specified number of divisions and then recombines them in the order specified (most significant division = 0,least = number divisions-1)
      mask init:
      | munge_init(gcb, ...
      |     'divisions', divisions, ...
      |     'div_size', div_size, ...
      |     'order', order, ...
      |     'arith_type_out', arith_type_out, ...
      |     'bin_pt_out', bin_pt_out);
      settings: AttributesFormatString=|
      | split:32
      | join:0
      | Unsigned [32,0]
      mask TypeOptions arith_type_out: Unsigned | Signed  (2's comp) | Floating-point
  data_out : Outport
  wires:
  convert_addr/1 -> casper_library_scopes_snap_circ_bram_addr/1
  convert_din1/1 -> casper_library_scopes_snap_circ_bram_data_in/1
  data_in/1 -> munge_in/1(din)
  calc_add/1(out) -> convert_addr/1
  casper_library_scopes_snap_circ_bram_we/1 -> mem/3(In3)
  casper_library_scopes_snap_circ_bram_data_in/1 -> mem/2(In2)
  casper_library_scopes_snap_circ_bram_addr/1 -> mem/1(In1)
  convert_we/1 -> casper_library_scopes_snap_circ_bram_we/1
  casper_library_scopes_snap_circ_bram_data_out/1 -> munge_out/1(din)
  mem/1(Out1) -> casper_library_scopes_snap_circ_bram_data_out/1
  addr/1 -> calc_add/1(in)
  we/1 -> convert_we/1
  munge_out/1(dout) -> data_out/1
  munge_in/1(dout) -> convert_din1/1
